simulink model "ecu_egrpos"  (R2026a)
settings: Solver=FixedStepDiscrete  StopTime=10  FixedStep=0.001  SampleTimeConstraint=STIndependent
Description:
  | EGR valve position PID. Source of truth for firmware/gen/ecu_egrpos.
settings Model: Creator=jj1001000  LastModifiedBy=jj1001000
settings OptimizationCC: DefaultUnderspecifiedDataType=single
settings DebuggingCC: ParameterPrecisionLossMsg=none
settings HardwareCC: ProdLargestAtomicInteger=Long  ProdLargestAtomicFloat=Double  ProdHWDeviceType=ARM Compatible->ARM Cortex-M
settings RTWCC: SystemTargetFile=ert.tlc  GenCodeOnly=on  Description=Embedded Coder
settings ERTTargetCC: UtilityFuncGeneration=Shared location  IncludeMdlTerminateFcn=off  CodeInterfacePackaging=Reusable function  SupportNonFinite=off

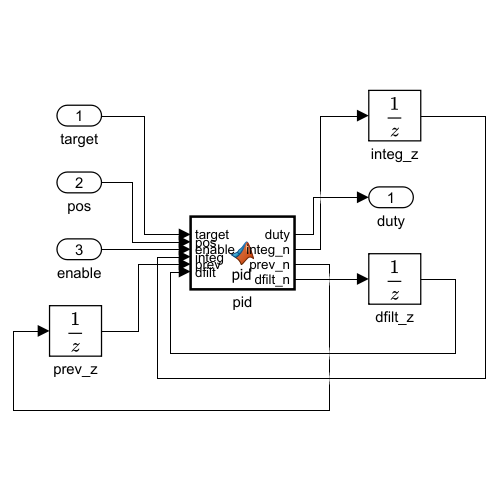
[thumbnail: Simulink's stored preview of the top-level diagram]
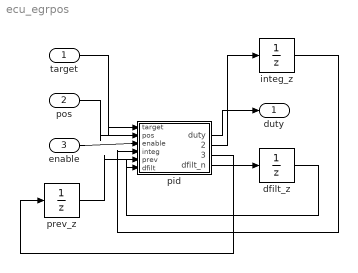
== system ecu_egrpos ==
  target : Inport  OutDataTypeStr=single
  pos : Inport  Port=2  OutDataTypeStr=single
  enable : Inport  Port=3  OutDataTypeStr=uint8
  dfilt_z : UnitDelay  SampleTime=-1
  integ_z : UnitDelay  SampleTime=-1
  pid : MATLAB Function  TreatAsAtomicUnit=on
  prev_z : UnitDelay  SampleTime=-1
  duty : Outport  OutDataTypeStr=single
  wires:
  pid/1(duty) -> duty/1
  pos/1 -> pid/2(pos)
  target/1 -> pid/1(target)
  enable/1 -> pid/3(enable)
  prev_z/1 -> pid/5(prev)
  pid/4(dfilt_n) -> dfilt_z/1
  dfilt_z/1 -> pid/6(dfilt)
  pid/3(prev_n) -> prev_z/1
  pid/2(integ_n) -> integ_z/1
  integ_z/1 -> pid/4(integ)

== matlab function ecu_egrpos/pid ==
  data: target input single; duty output single; pos input single; enable input uint8; integ input single; prev input single; dfilt input single; integ_n output single; prev_n output single; dfilt_n output single
function [duty, integ_n, prev_n, dfilt_n] = pid(target, pos, enable, integ, prev, dfilt)
%#codegen
dpos = (pos - prev) / single(0.00100000005);
prev_n = pos;
if enable == 0 || target <= single(2)          % coast: the spring closes it
    integ_n = single(0); dfilt_n = single(0); duty = single(0);
    return
end
dfilt_n = dfilt + single(0.100000001) * (dpos - dfilt);
err = target - pos;
out = single(0.0199999996) * err + integ - single(0.000500000024) * dfilt_n;
integ_n = integ;
if ~((out >= single(0.949999988) && err > single(0)) || (out <= single(-0.949999988) && err < single(0)))
    integ_n = sat(integ + single(0.100000001) * err * single(0.00100000005), single(-0.949999988), single(0.949999988));
end
duty = sat(single(0.0199999996) * err + integ_n - single(0.000500000024) * dfilt_n, single(-0.949999988), single(0.949999988));
end

function y = sat(x, lo, hi)
if x < lo
    y = lo;
elseif x > hi
    y = hi;
else
    y = x;
end
end
